simulink model "Dynamics_CNC"  (R2026a)
settings: Solver=ode4  StopTime=20  FixedStep=1e-3
settings Model: Creator=tomas_w6j1h7m  LastModifiedBy=tomas_w6j1h7m

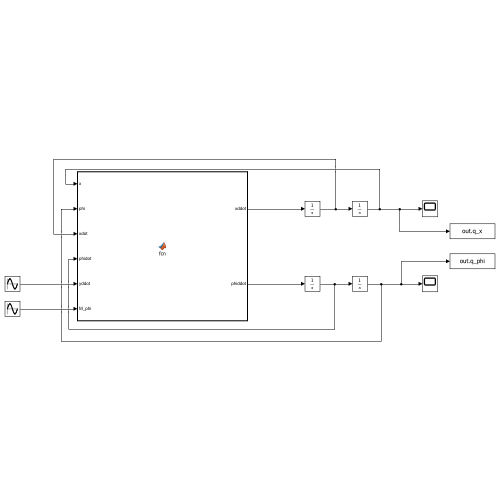
[thumbnail: Simulink's stored preview of the top-level diagram]
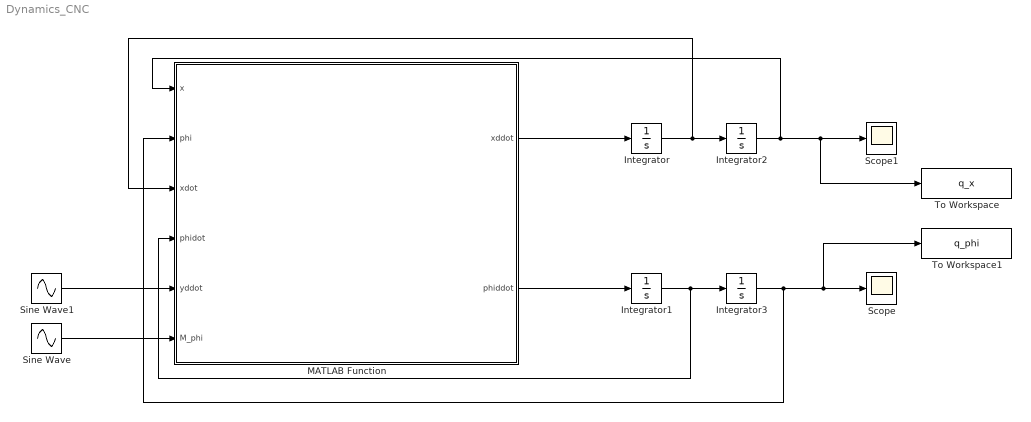
== system Dynamics_CNC ==
  Integrator : Integrator
  Integrator1 : Integrator
  Integrator2 : Integrator  InitialCondition=0.1
  Integrator3 : Integrator  InitialCondition=-pi/4
  MATLAB Function : MATLAB Function  TreatAsAtomicUnit=on
  Scope : Scope
      settings: ActiveDisplayYMinimum=-3.5567992621975297  ActiveDisplayYMaximum=0.70838578164525046
  Scope1 : Scope
      settings: ActiveDisplayYMinimum=0.020541308228781585  ActiveDisplayYMaximum=0.8151282259409659
  Sine Wave : Sin  Amplitude=120  Frequency=3  SampleTime=0
  Sine Wave1 : Sin  Amplitude=-20  Frequency=10  SampleTime=0
  To Workspace : ToWorkspace  VariableName=q_x  SampleTime=-1
  To Workspace1 : ToWorkspace  VariableName=q_phi  SampleTime=-1
  wires:
  MATLAB Function/1(xddot) -> Integrator/1
  MATLAB Function/2(phiddot) -> Integrator1/1
  Integrator1/1 -> Integrator3/1, MATLAB Function/4(phidot)
  Integrator/1 -> Integrator2/1, MATLAB Function/3(xdot)
  Integrator2/1 -> To Workspace/1, Scope1/1, MATLAB Function/1(x)
  Integrator3/1 -> To Workspace1/1, Scope/1, MATLAB Function/2(phi)
  Sine Wave/1 -> MATLAB Function/6(M_phi)
  Sine Wave1/1 -> MATLAB Function/5(yddot)

== matlab function Dynamics_CNC/MATLAB Function ==
  data: x input; xddot output; phi input; xdot input; phidot input; yddot input; M_phi input; phiddot output
function [xddot,phiddot] = fcn(x,phi,xdot,phidot,yddot,M_phi)

%% Parameters from Table 1

J_h2    = 1.2;
L23     = 0.05;
d_PD    = 10;
d_phi   = 2;
d_x     = 0.5;
g        = 9.81;
k_PD     = 380;
k_phi    = 100;
m_c      = 2;
m_h      = 0.7;
phi_h3   = pi/3;
phi_ref  = -pi/2;
x_PDref  = 0.5;

%% Defining the EoM

[M,rhs] = EOM_Function( ...
    J_h2,L23,M_phi,d_PD,d_phi,d_x,g,...
    k_PD,k_phi,m_c,m_h,...
    phi,phi_h3,phidot,phi_ref,...
    x,x_PDref,xdot,yddot);

qdd = M\rhs;

xddot   = qdd(1);
phiddot = qdd(2);

end
